simulink model "testDiscreteTower"  (R2019b)
settings: Solver=FixedStepAuto  StartTime=0.0  StopTime=10.0  FixedStep=DT  RelTol=1e-3
values from neighbouring files (symbols this model uses):
  Asw_z = ss_sw_disc.A    [calcDiscretParamTowerMotion.m]
  Bsw_z = ss_sw_disc.B    [calcDiscretParamTowerMotion.m]
  DT = 0.008    [dataDLR.m]    (also in generateReport.m; initLPVParam.m; initWorkspace.m; runCalculateEvalCriteria.m)
  wecs = 3.0    [DD_test.sldd]    (also in dataDLR.m = struct; testOutList.m = struct; testqLPV.m = struct)
settings Model: DataDictionary=DD_Mdl.sldd  Creator=ditt_aj  LastModifiedBy=ditt_aj

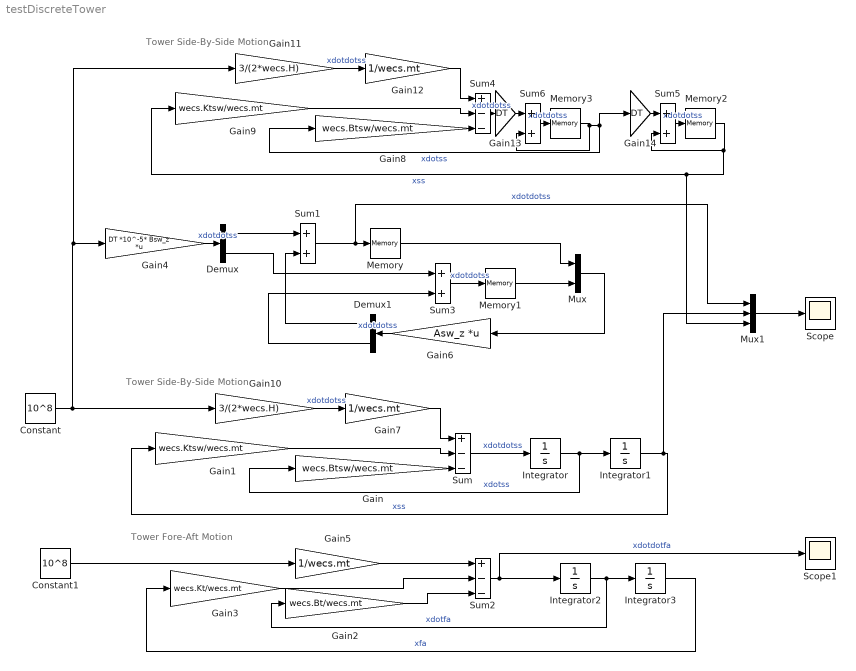
== system testDiscreteTower ==
  note: Tower Fore-Aft Motion
  note: Tower Side-By-Side Motion
  note: Tower Side-By-Side Motion
  Constant : Constant  Value=10^8
  Constant1 : Constant  Value=10^8
  Demux : Demux  Outputs=2
  Demux1 : Demux  Outputs=2
  Gain : Gain  Gain=wecs.Btsw/wecs.mt
  Gain1 : Gain  Gain=wecs.Ktsw/wecs.mt
  Gain10 : Gain  Gain=3/(2*wecs.H)
  Gain11 : Gain  Gain=3/(2*wecs.H)
  Gain12 : Gain  Gain=1/wecs.mt
  Gain13 : Gain  Gain=DT
  Gain14 : Gain  Gain=DT
  Gain2 : Gain  Gain=wecs.Bt/wecs.mt
  Gain3 : Gain  Gain=wecs.Kt/wecs.mt
  Gain4 : Gain  Gain=DT *10^-5* Bsw_z  Multiplication=Matrix(K*u)
  Gain5 : Gain  Gain=1/wecs.mt
  Gain6 : Gain  Gain=Asw_z  Multiplication=Matrix(K*u)
  Gain7 : Gain  Gain=1/wecs.mt
  Gain8 : Gain  Gain=wecs.Btsw/wecs.mt
  Gain9 : Gain  Gain=wecs.Ktsw/wecs.mt
  Integrator{,1..3} (4 alike) : Integrator
  Memory{,1..3} (4 alike) : Memory
  Mux : Mux  Inputs=2
  Mux1 : Mux  Inputs=3
  Scope : Scope
  Scope1 : Scope
  Sum : Sum  Inputs=+--
  Sum{1,3,5..6} (4 alike) : Sum
  Sum2 : Sum  Inputs=+--
  Sum4 : Sum  Inputs=+--
  wires:
  Gain10/1 -> Gain7/1  "xdotdotss"
  Integrator1/1 -> Mux1/2, Gain1/1  "xss"
  Gain1/1 -> Sum/2
  Integrator/1 -> Integrator1/1, Gain/1  "xdotss"
  Sum/1 -> Integrator/1  "xdotdotss"
  Sum2/1 -> Scope1/1, Integrator2/1  "xdotdotfa"
  Gain7/1 -> Sum/1
  Integrator2/1 -> Gain2/1, Integrator3/1  "xdotfa"
  Gain3/1 -> Sum2/2
  Constant1/1 -> Gain5/1
  Integrator3/1 -> Gain3/1  "xfa"
  Gain/1 -> Sum/3
  Gain2/1 -> Sum2/3
  Gain5/1 -> Sum2/1
  Sum1/1 -> Mux1/1, Memory/1  "xdotdotss"
  Gain4/1 -> Demux/1  "xdotdotss"
  Demux/1 -> Sum1/1
  Memory1/1 -> Mux/2
  Mux/1 -> Gain6/1
  Sum3/1 -> Memory1/1  "xdotdotss"
  Gain6/1 -> Demux1/1  "xdotdotss"
  Demux1/1 -> Sum1/2
  Demux/2 -> Sum3/1
  Demux1/2 -> Sum3/2
  Mux1/1 -> Scope/1
  Memory/1 -> Mux/1
  Constant/1 -> Gain11/1, Gain4/1, Gain10/1
  Gain12/1 -> Sum4/1
  Gain8/1 -> Sum4/3
  Gain9/1 -> Sum4/2
  Memory3/1 -> Gain14/1, Gain8/1, Sum6/2  "xdotss"
  Memory2/1 -> Mux1/3, Gain9/1, Sum5/2  "xss"
  Gain11/1 -> Gain12/1  "xdotdotss"
  Sum4/1 -> Gain13/1  "xdotdotss"
  Sum5/1 -> Memory2/1  "xdotdotss"
  Gain13/1 -> Sum6/1
  Sum6/1 -> Memory3/1  "xdotdotss"
  Gain14/1 -> Sum5/1
